simulink model "copilot_closed_loop_broken"  (R2026b)
settings: Solver=ode45  StopTime=simulationStopTime_demo  FixedStep=0.002  EnableMultiTasking=on
undefined symbols (not defined in the file or in its folder): Kp_missing
settings Model: Creator=ecosgrov  LastModifiedBy=garellan
settings SolverCC: PositivePriorityOrder=on
settings DataIOCC: ReturnWorkspaceOutputs=off
settings DebuggingCC: ArithmeticOperatorsInVariantConditions=warning
settings SFSimCC: CustomCodeUndefinedFunction=UseInterfaceOnly  SimUseLocalCustomCode=off
settings RTWCC: RTWUseLocalCustomCode=off
settings CodeAppCC: StateflowObjectComments=on
settings ConfigComp: CovMetricSettings=ds

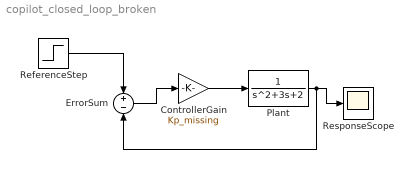
== system copilot_closed_loop_broken ==
  ControllerGain : Gain  Gain=Kp_missing
  ErrorSum : Sum  Inputs=+-
  Plant : TransferFcn  Denominator=[1 3 2]
  ReferenceStep : Step  Time=0  FinalValue=stepAmplitude_demo  SampleTime=0
  ResponseScope : Scope
  wires:
  Plant/1 -> ResponseScope/1, ErrorSum/2
  ControllerGain/1 -> Plant/1
  ErrorSum/1 -> ControllerGain/1
  ReferenceStep/1 -> ErrorSum/1
